simulink model "aproximacion_peaje"  (R2025b)
settings: Solver=ode45  StartTime=0.0  StopTime=tSim  MaxStep=0.05  RelTol=1e-6
values from neighbouring files (symbols this model uses):
  a = q.a * p.factor_a    [aproximacion_ode45.m]    (also in motor_inicializar.m; validar_simulink.m)
  b = q.b * p.factor_b    [aproximacion_ode45.m]    (also in motor_inicializar.m; validar_simulink.m)
  T = q.T * p.factor_T    [aproximacion_ode45.m]    (also in fase2_demo.m = R.vehiculos; motor_inicializar.m; validar_simulink.m)
  v0 = q.v0 * p.factor_v0    [aproximacion_ode45.m]    (also in motor_inicializar.m; validar_simulink.m)
undefined symbols (not defined in the file or in its folder): aMax, s0, v_ini, xObs
settings Model: Creator=WebMaster  LastModifiedBy=WebMaster

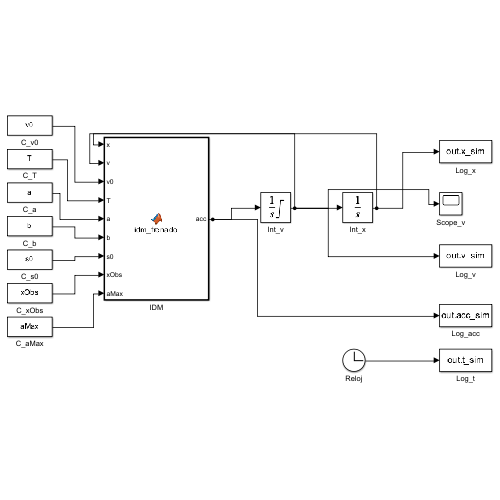
[thumbnail: Simulink's stored preview of the top-level diagram]
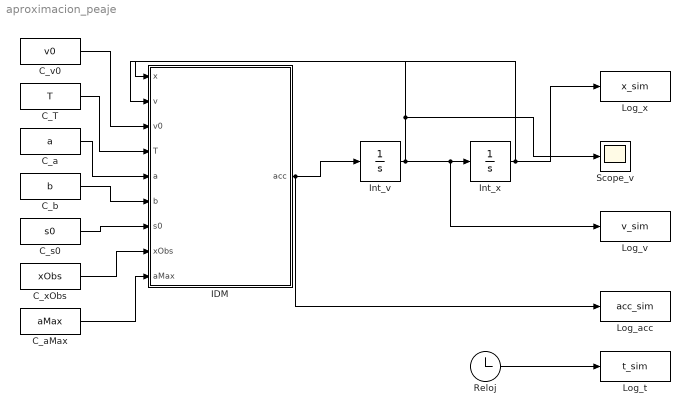
== system aproximacion_peaje ==
  C_T : Constant  Value=T
  C_a : Constant  Value=a
  C_aMax : Constant  Value=aMax
  C_b : Constant  Value=b
  C_s0 : Constant  Value=s0
  C_v0 : Constant  Value=v0
  C_xObs : Constant  Value=xObs
  IDM : MATLAB Function  TreatAsAtomicUnit=on
  Int_v : Integrator  InitialCondition=v_ini  LimitOutput=on  LowerSaturationLimit=0
  Int_x : Integrator
  Log_acc : ToWorkspace  VariableName=acc_sim  SampleTime=-1
  Log_t : ToWorkspace  VariableName=t_sim  SampleTime=-1
  Log_v : ToWorkspace  VariableName=v_sim  SampleTime=-1
  Log_x : ToWorkspace  VariableName=x_sim  SampleTime=-1
  Reloj : Clock
  Scope_v : Scope
  wires:
  C_v0/1 -> IDM/3(v0)
  C_T/1 -> IDM/4(T)
  C_a/1 -> IDM/5(a)
  C_b/1 -> IDM/6(b)
  C_s0/1 -> IDM/7(s0)
  C_xObs/1 -> IDM/8(xObs)
  C_aMax/1 -> IDM/9(aMax)
  IDM/1(acc) -> Int_v/1, Log_acc/1
  Int_v/1 -> Int_x/1, Log_v/1, IDM/2(v), Scope_v/1
  Int_x/1 -> IDM/1(x), Log_x/1
  Reloj/1 -> Log_t/1

== matlab function aproximacion_peaje/IDM ==
  data: x input; acc output; v input; v0 input; T input; a input; b input; s0 input; xObs input; aMax input
function acc = idm_frenado(x, v, v0, T, a, b, s0, xObs, aMax)
% Modelo de Conductor Inteligente frente a un obstáculo detenido en xObs
s = max(xObs - x, 0.01);
sEst = s0 + max(0, v*T + v*v/(2*sqrt(a*b)));
acc = a*(1 - (v/v0)^4 - (sEst/s)^2);
acc = max(acc, -aMax);
